simulink model "tg9"  (R2022a)
settings: Solver=ode15s  StartTime=0.0  StopTime=10  MaxStep=0.01  RelTol=1e-3
InitFcn:
  | mecha_param2
  | control_param0
values from neighbouring files (symbols this model uses):
  b0 = 0    [sim_IMMC.m]
  b1 = 1    [sim_IMMC.m]
  back0 = 0    [sim_IMMC.m]
  back1 = 0    [sim_IMMC.m]
  boff = 0    [sim_IMMC.m]
  bon = 0    [sim_IMMC.m]
  c = 0.05    [mecha_param2.m]
  c_jointstop = 0.3 / (pi/180)    (= 17.1887338539)    [mecha_param2.m]
  calctalus = sqrt((L_foot - (DJ1x_foot))^2 + (H_foot-r_cs)^2)    [mecha_param2.m]
  calctoes = sqrt((H_foot-r_cs)^2 + (DJ1x_foot)^2)    [mecha_param2.m]
  corrD = 0.001    [control_param0.m]
  DG_HAT = 0.35    [mecha_param2.m]
  DG_thigh = 0.28    [mecha_param2.m]
  DJ1x_foot = 0.16-r_cs    (= 0.135)    [mecha_param2.m]
  eref = 0.04    [mecha_param2.m]
  FmaxBFSH = 350    [mecha_param2.m]
  FmaxGAS = 1500    [mecha_param2.m]
  FmaxGLU = 1500    [mecha_param2.m]
  FmaxHAM = 3000    [mecha_param2.m]
  FmaxHFL = 2000    [mecha_param2.m]
  FmaxRF = 1200    [mecha_param2.m]
  FmaxSOL = 4000    [mecha_param2.m]
  FmaxTA = 800    [mecha_param2.m]
  FmaxVAS = 6000    [mecha_param2.m]
  g = 9.81    [mecha_param2.m]
  g0 = 0    [sim_IMMC.m]
  g1 = 0    [sim_IMMC.m]
  H_foot = 0.08    [mecha_param2.m]
  In_HAT = 3    [mecha_param2.m]
  In_shank = 0.05    [mecha_param2.m]
  In_thigh = 0.15    [mecha_param2.m]
  K = 5    [mecha_param2.m]
  knee_thigh = [0 0 -(L_thigh/2)]    [mecha_param2.m]
  Kpress = m_HAT * g / DeltaThRef    (= 104967)    [mecha_param2.m]
  L_foot = 0.2    [mecha_param2.m]
  L_HAT = 0.8    [mecha_param2.m]
  L_shank = 0.46    [mecha_param2.m]
  L_thigh = 0.46    [mecha_param2.m]
  LoHAM = table2array(mt('LoHAM', 1))    [control_param0.m]
  LoHFL = table2array(mt('LoHFL', 1))    [control_param0.m]
  longD = longD - corrD    (= 0.019)    [control_param0.m]
  loptBFSH = 0.12    [mecha_param2.m]
  loptGAS = 0.05    [mecha_param2.m]
  loptGLU = 0.11    [mecha_param2.m]
  loptHAM = 0.10    (= 0.1)    [mecha_param2.m]
  loptHFL = 0.11    [mecha_param2.m]
  loptRF = 0.08    [mecha_param2.m]
  loptSOL = 0.04    [mecha_param2.m]
  loptTA = 0.06    [mecha_param2.m]
  loptVAS = 0.08    [mecha_param2.m]
  LoTA = table2array(mt('LoTA', 1))    [control_param0.m]
  lslackBFSH = 0.10    (= 0.1)    [mecha_param2.m]
  lslackGAS = 0.40    (= 0.4)    [mecha_param2.m]
  lslackGLU = 0.13    [mecha_param2.m]
  lslackHAM = 0.31    [mecha_param2.m]
  lslackHFL = 0.10    (= 0.1)    [mecha_param2.m]
  lslackRF = 0.35    [mecha_param2.m]
  lslackSOL = 0.26    [mecha_param2.m]
  lslackTA = 0.24    [mecha_param2.m]
  lslackVAS = 0.23    [mecha_param2.m]
  m_HAT = 53.5    [mecha_param2.m]
  m_shank = 3.5    [mecha_param2.m]
  m_thigh = 8.5    [mecha_param2.m]
  midD = midD - corrD    (= 0.009)    [control_param0.m]
  N = 1.5    [mecha_param2.m]
  nonoff = 0    [control_param0.m]
  phi_a_low = (70) * (pi / 180)    (= 1.2217304764)    [mecha_param2.m]
  phi_a_up = (130) * (pi / 180)    (= 2.26892802759)    [mecha_param2.m]
  phi_dl = 180    [mecha_param2.m]
  phi_h = 230 * (pi / 180)    (= 4.01425727959)    [mecha_param2.m]
  phi_k = 175 * (pi / 180)    (= 3.05432619099)    [mecha_param2.m]
  phictoes = asind((DJ1y_foot-r_cs)/calctoes)    [mecha_param2.m]
  phimaxGASa = 100*pi/180    (= 1.74532925199)    [mecha_param2.m]
  phimaxGASk = 140*pi/180    (= 2.44346095279)    [mecha_param2.m]
  phimaxRFk = 165*pi/180    (= 2.87979326579)    [mecha_param2.m]
  phimaxSOL = 100*pi/180    (= 1.74532925199)    [mecha_param2.m]
  phimaxTA = 80*pi/180    (= 1.3962634016)    [mecha_param2.m]
  phimaxVAS = 165*pi/180    (= 2.87979326579)    [mecha_param2.m]
  phirefBFSH = 160*pi/180    (= 2.79252680319)    [mecha_param2.m]
  phirefGASa = 80*pi/180    (= 1.3962634016)    [mecha_param2.m]
  phirefGASk = 165*pi/180    (= 2.87979326579)    [mecha_param2.m]
  phirefGLU = 120*pi/180    (= 2.09439510239)    [mecha_param2.m]
  phirefHAMh = 150*pi/180    (= 2.61799387799)    [mecha_param2.m]
  phirefHAMk = 180*pi/180    (= 3.14159265359)    [mecha_param2.m]
  phirefHFL = 160*pi/180    (= 2.79252680319)    [mecha_param2.m]
  phirefRFh = 170*pi/180    (= 2.96705972839)    [mecha_param2.m]
  phirefRFk = 125*pi/180    (= 2.18166156499)    [mecha_param2.m]
  phirefSOL = 90*pi/180    (= 1.57079632679)    [mecha_param2.m]
  phirefTA = 110*pi/180    (= 1.91986217719)    [mecha_param2.m]
  phirefVAS = 120*pi/180    (= 2.09439510239)    [mecha_param2.m]
  phiScaleGASa = acos(rGASamin/rGASamax)/(phiminGASa-phimaxGASa)    [mecha_param2.m]
  phiScaleGASk = acos(rGASkmin/rGASkmax)/(phiminGASk-phimaxGASk)    [mecha_param2.m]
  phiScaleRFk = acos(rRFkmin/rRFkmax)/(phiminRFk-phimaxRFk)    [mecha_param2.m]
  phiScaleSOL = acos(rSOLmin/rSOLmax)/(phiminSOL-phimaxSOL)    [mecha_param2.m]
  phiScaleTA = acos(rTAmin/rTAmax)/(phiminTA-phimaxTA)    [mecha_param2.m]
  phiScaleVAS = acos(rVASmin/rVASmax)/(phiminVAS-phimaxVAS)    [mecha_param2.m]
  r1 = 0    [sim_IMMC.m]
  r_cs = 0.025    [mecha_param2.m]
  rBFSH = 0.04    [mecha_param2.m]
  rGASamax = 0.06    [mecha_param2.m]
  rGASkmax = 0.05    [mecha_param2.m]
  rGLU = 0.08    [mecha_param2.m]
  rHAMh = 0.08    [mecha_param2.m]
  rHAMk = 0.05    [mecha_param2.m]
  rHFL = 0.08    [mecha_param2.m]
  rhoBFSH = 0.7    [mecha_param2.m]
  rhoGASa = 0.7    [mecha_param2.m]
  rhoGASk = 0.7    [mecha_param2.m]
  rhoGLU = 0.5    [mecha_param2.m]
  rhoHAMh = 0.5    [mecha_param2.m]
  rhoHAMk = 0.5    [mecha_param2.m]
  rhoHFL = 0.5    [mecha_param2.m]
  rhoRFh = 0.3    [mecha_param2.m]
  rhoRFk = 0.5    [mecha_param2.m]
  rhoSOL = 0.5    [mecha_param2.m]
  rhoTA = 0.7    [mecha_param2.m]
  rhoVAS = 0.6    [mecha_param2.m]
  rRFh = 0.08    [mecha_param2.m]
  rRFkmax = 0.06    [mecha_param2.m]
  rSOLmax = 0.06    [mecha_param2.m]
  ... (+25 more)
undefined symbols (not defined in the file or in its folder): beta11, beta12, beta13, beta14, beta15, beta16, beta21, beta22, beta23, beta24, beta25, beta26, beta31, beta32, beta33, beta34, beta35, beta36, beta41, beta42, beta43, beta44, beta45, beta46, beta51, beta52, beta53, beta54, beta55, beta56, betab1, betab2, betab3, betab4, betab5, betab6, betap11, betap12, betap13, betap14, betap15, betap16, betap21, betap22, betap23, betap24, betap25, betap26, betap31, betap32, betap33, betap34, betap35, betap36, betap41, betap42, betap43, betap44, betap45, betap46 ... (+102)
libraries: sm_lib x89, simulink x72, nesl_utility x58, simulink_extras x18
(part 11 of 12)

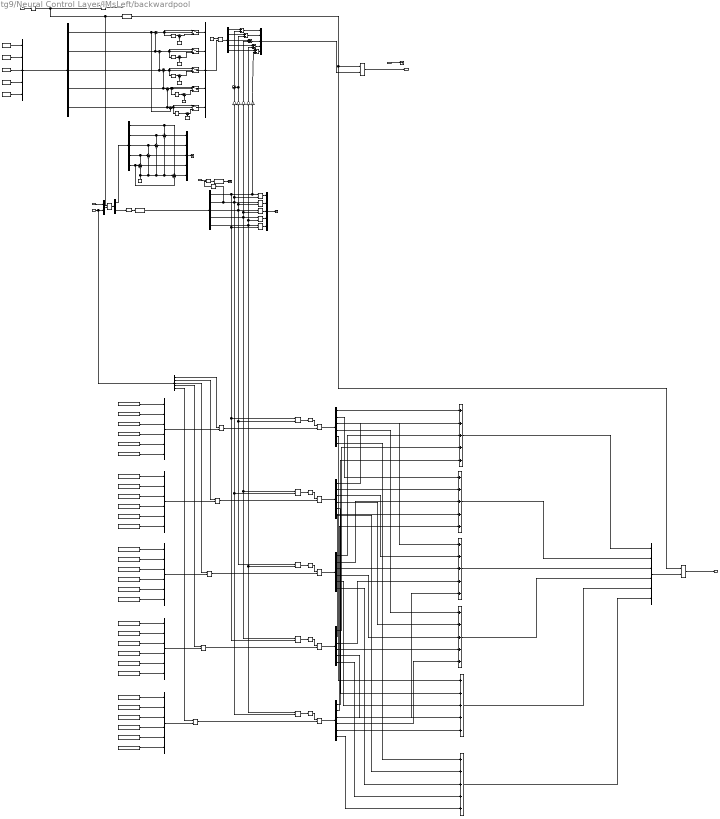
== system tg9/Neural Control Layer/IMsLeft/backwardpool ==
  eta : Inport
  phase : Inport  Port=2
  ui : Inport  Port=3
  right2left : Inport  Port=4
  triggers : Inport  Port=5
  control : Inport  Port=6
  Abs{,1..4} (5 alike) : Abs  ZeroCross=off  SaturateOnIntegerOverflow=off
  Add{,1..4} (5 alike) : Sum
  Add{5,11..15} (6 alike) : Sum  Inputs=+++++
  Cast To Double : DataTypeConversion  OutDataTypeStr=double  SaturateOnIntegerOverflow=off  RndMeth=Floor
  Cast To Double1 : DataTypeConversion  OutDataTypeStr=double  SaturateOnIntegerOverflow=off  RndMeth=Floor
  Cast To Double2 : DataTypeConversion  OutDataTypeStr=double  SaturateOnIntegerOverflow=off  RndMeth=Floor
  Compare To Constant : simulink/Logic and Bit Operations/Compare To Constant  relop=>  const=0.001  OutDataTypeStr=boolean  ZeroCross=off
  Compare To Constant1 : simulink/Logic and Bit Operations/Compare To Constant  relop=<  const=1  OutDataTypeStr=boolean  ZeroCross=off
  Compare To Zero1 : simulink/Logic and Bit Operations/Compare To Zero  relop=>  OutDataTypeStr=boolean  ZeroCross=off
  Constant1 : Constant
  Constant{2,4..6,10} (5 alike) : Constant  Value=2
  Constant3 : Constant  Value=pi
  Demux{,1,4..6} (5 alike) : Demux  Outputs=5
  Demux{8..12} (5 alike) : Demux  Outputs=6
  Demux3 : Demux  Outputs=2
  Divide : Product  Inputs=*/
  Gain{1..4,45} (5 alike) : Gain  Gain=10
  IsPositive{6..10} (5 alike) : simulink/Logic and Bit Operations/Compare To Zero  relop===  OutDataTypeStr=uint8  ZeroCross=off
  Logical Operator : Logic  AllPortsSameDT=off  OutDataTypeStr=boolean
  Mux{1..3,6..7} (5 alike) : Mux  Inputs=5
  Mux{10,16..20} (6 alike) : Mux  Inputs=6
  Mux5 : Mux  Inputs=2
  Product{1..3,6,9,12,17..29,32..36} (24 alike) : Product
  Sum{,1..3,5..6,8..9,11..12} (10 alike) : Sum  Inputs=|-+
  Sum{4,7,10,13} (4 alike) : Sum  Inputs=-+-
  Sum14 : Sum  Inputs=+--
  Sum15 : Sum  Inputs=|++
  Switch{,1..4} (5 alike) : Switch  Criteria=u2 > Threshold  ZeroCross=off  SaturateOnIntegerOverflow=off  InputSameDT=off
  Terminator{,2..4} (4 alike) : Terminator
  betap11 : Constant  Value=betap11
  betap12 : Constant  Value=betap12
  betap13 : Constant  Value=betap13
  betap14 : Constant  Value=betap14
  betap15 : Constant  Value=betap15
  betap16 : Constant  Value=betap16
  betap21 : Constant  Value=betap21
  betap22 : Constant  Value=betap22
  betap23 : Constant  Value=betap23
  betap24 : Constant  Value=betap24
  betap25 : Constant  Value=betap25
  betap26 : Constant  Value=betap26
  betap31 : Constant  Value=betap31
  betap32 : Constant  Value=betap32
  betap33 : Constant  Value=betap33
  betap34 : Constant  Value=betap34
  betap35 : Constant  Value=betap35
  betap36 : Constant  Value=betap36
  betap41 : Constant  Value=betap41
  betap42 : Constant  Value=betap42
  betap43 : Constant  Value=betap43
  betap44 : Constant  Value=betap44
  betap45 : Constant  Value=betap45
  betap46 : Constant  Value=betap46
  betap51 : Constant  Value=betap51
  betap52 : Constant  Value=betap52
  betap53 : Constant  Value=betap53
  betap54 : Constant  Value=betap54
  betap55 : Constant  Value=betap55
  betap56 : Constant  Value=betap56
  theta1 : Constant  Value=thetab1
  theta2 : Constant  Value=thetab2
  theta3 : Constant  Value=thetab3
  theta4 : Constant  Value=thetab4
  theta5 : Constant  Value=thetab5
  vartheta : Outport
  beta : Outport  Port=2
  trigger_out : Outport  Port=3
  wires:
  Sum7/1 -> Mux2/2
  Demux4/4 -> Sum9/1, Sum6/2
  Sum15/1 -> Add/2
  Add2/1 -> Mux7/5
  Switch4/1 -> Mux1/5
  Demux/1 -> Sum14/1, Sum4/1
  Sum3/1 -> Switch/3
  Sum4/1 -> Mux2/1
  Demux/5 -> Sum13/2, Sum14/3
  Abs1/1 -> Sum1/1
  Demux5/4 -> Add4/1
  Mux7/1 -> Product17/2
  Sum8/1 -> Switch3/3
  Sum1/1 -> Switch1/3
  Constant1/1 -> Divide/1
  Sum2/1 -> Abs1/1, Switch1/1, Switch1/2
  Switch/1 -> Mux1/1
  Constant2/1 -> Sum3/2
  Constant5/1 -> Sum5/2
  Demux3/1 -> Demux/1
  Sum11/1 -> Switch4/3
  Abs2/1 -> Sum5/1
  Switch2/1 -> Mux1/3
  Constant3/1 -> Sum14/2, Sum4/3, Sum7/3, Sum10/3, Sum13/3
  Demux4/3 -> Sum2/2, Sum6/1
  Sum12/1 -> Switch4/1, Abs4/1, Switch4/2
  Product2/1 -> Mux3/2
  Sum14/1 -> Mux2/5
  Demux5/1 -> Add/1
  Demux/3 -> Sum7/2, Sum10/1
  Sum5/1 -> Switch2/3
  Compare To Zero1/1 -> Product19/2, Cast To Double2/1, Product18/1
  Product18/1 -> Demux3/1
  Product12/1 -> Mux3/5
  triggers/1 -> Product19/1
  Cast To Double/1 -> Demux1/1
  Demux/2 -> Sum4/2, Sum7/1
  phase/1 -> Mux5/1
  Abs3/1 -> Sum8/1
  Sum6/1 -> Switch2/2, Switch2/1, Abs2/1
  Sum13/1 -> Mux2/4
  Constant6/1 -> Sum11/2
  Logical Operator/1 -> Cast To Double1/1
  ui/1 -> Demux6/1, Mux5/2
  Demux5/3 -> Add3/1
  Demux5/2 -> Add1/1
  Demux5/5 -> Add2/1
  Mux1/1 -> Divide/2
  Demux4/5 -> Sum12/1, Sum9/2
  Demux4/2 -> Sum2/1, Sum/2
  Gain1/1 -> Sum15/2, Add1/2
  Add1/1 -> Mux7/2
  Cast To Double1/1 -> Terminator2/1
  Add/1 -> Mux7/1
  right2left/1 -> Logical Operator/1
  Compare To Constant1/1 -> Logical Operator/2
  Constant4/1 -> Sum1/2
  Demux3/2 -> Compare To Constant/1
  Sum/1 -> Switch/2, Abs/1, Switch/1
  Abs4/1 -> Sum11/1
  eta/1 -> Terminator4/1
  Product1/1 -> Mux3/1
  Mux5/1 -> Product18/2
  Abs/1 -> Sum3/1
  Compare To Constant/1 -> Cast To Double/1
  Switch3/1 -> Mux1/4
  Demux4/1 -> Sum/1, Sum12/2
  Sum9/1 -> Abs3/1, Switch3/2, Switch3/1
  Constant10/1 -> Sum8/2
  Product17/1 -> vartheta/1
  Product9/1 -> Mux3/4
  Divide/1 -> Demux5/1
  Product6/1 -> Mux3/3
  Sum10/1 -> Mux2/3
  Cast To Double2/1 -> Product29/1, Product17/1
  control/1 -> Compare To Zero1/1
  Gain4/1 -> Add2/2
  Product19/1 -> trigger_out/1
  Mux6/1 -> Demux4/1
  Demux/4 -> Sum13/1, Sum10/2
  Switch1/1 -> Mux1/2
  Add3/1 -> Mux7/3
  Add4/1 -> Mux7/4
  Gain2/1 -> Add4/2
  Gain45/1 -> Add3/2
  Mux2/1 -> Terminator/1
  Mux3/1 -> Terminator3/1
  Gain3/1 -> Sum15/1
  theta5/1 -> Mux6/5
  theta4/1 -> Mux6/4
  theta3/1 -> Mux6/3
  theta2/1 -> Mux6/2
  theta1/1 -> Mux6/1
  betap11/1 -> Mux10/1
  Demux1/3 -> Product22/1, Product25/2, Product6/1, Product2/2, Gain1/1
  Demux1/2 -> Product2/1, Product28/2, Product3/2, Product1/2, Gain3/1, Compare To Constant1/1
  Product26/1 -> Demux8/1
  IsPositive7/1 -> Product26/1
  Product25/1 -> IsPositive7/1
  betap12/1 -> Mux10/2
  betap13/1 -> Mux10/3
  betap14/1 -> Mux10/4
  betap16/1 -> Mux10/6
  betap15/1 -> Mux10/5
  Product3/1 -> IsPositive6/1
  IsPositive6/1 -> Product20/1
  Product20/1 -> Demux9/1
  Product21/1 -> Demux10/1
  Mux17/1 -> Product34/2
  IsPositive8/1 -> Product21/1
  Product22/1 -> IsPositive8/1
  Product24/1 -> IsPositive9/1
  IsPositive9/1 -> Product23/1
  Mux18/1 -> Product35/2
  Product23/1 -> Demux11/1
  Product27/1 -> Demux12/1
  Mux19/1 -> Product36/2
  IsPositive10/1 -> Product27/1
  Product28/1 -> IsPositive10/1
  Demux1/1 -> Product24/2, Product25/1, Product12/2, Product1/1, Gain4/1
  Demux1/4 -> Product9/1, Product24/1, Product3/1, Product6/2, Gain45/1
  Demux1/5 -> Product12/1, Product28/1, Product22/2, Product9/2, Gain2/1
  Demux8/1 -> Add5/1
  Demux9/2 -> Add11/2
  Demux10/3 -> Add12/3
  Demux11/4 -> Add13/4
  Demux12/5 -> Add14/5
  Demux8/2 -> Add11/1
  Demux8/3 -> Add12/1
  Demux8/4 -> Add13/1
  Demux8/5 -> Add14/1
  Demux8/6 -> Add15/1
  Demux9/1 -> Add5/2
  Demux9/3 -> Add12/2
  Demux9/4 -> Add13/2
  Demux9/5 -> Add14/2
  Demux9/6 -> Add15/2
  Demux10/1 -> Add5/3
  Demux10/2 -> Add11/3
  Demux10/4 -> Add13/3
  Demux10/5 -> Add14/3
  Demux10/6 -> Add15/3
  Demux11/1 -> Add5/4
  Demux11/2 -> Add11/4
  Demux11/3 -> Add12/4
  Demux11/5 -> Add14/4
  Demux11/6 -> Add15/4
  Demux12/1 -> Add5/5
  Demux12/2 -> Add11/5
  Demux12/3 -> Add12/5
  Demux12/4 -> Add13/5
  Demux12/6 -> Add15/5
  betap21/1 -> Mux16/1
  betap22/1 -> Mux16/2
  betap23/1 -> Mux16/3
  betap24/1 -> Mux16/4
  betap25/1 -> Mux16/5
  betap26/1 -> Mux16/6
  betap31/1 -> Mux17/1
  betap32/1 -> Mux17/2
  betap33/1 -> Mux17/3
  betap34/1 -> Mux17/4
  betap35/1 -> Mux17/5
  betap36/1 -> Mux17/6
  betap41/1 -> Mux18/1
  betap42/1 -> Mux18/2
  betap43/1 -> Mux18/3
  betap44/1 -> Mux18/4
  betap45/1 -> Mux18/5
  betap46/1 -> Mux18/6
  betap56/1 -> Mux19/6
  betap51/1 -> Mux19/1
  betap52/1 -> Mux19/2
  betap53/1 -> Mux19/3
  betap54/1 -> Mux19/4
  betap55/1 -> Mux19/5
  Add5/1 -> Mux20/1
  Add11/1 -> Mux20/2
  Add15/1 -> Mux20/6
  Add13/1 -> Mux20/4
  Add12/1 -> Mux20/3
  Add14/1 -> Mux20/5
  Mux10/1 -> Product32/2
  Product32/1 -> Product26/2
  Demux6/1 -> Product32/1
  Mux16/1 -> Product33/2
  Product33/1 -> Product20/2
  Demux6/2 -> Product33/1
  Product34/1 -> Product21/2
  Demux6/3 -> Product34/1
  Product35/1 -> Product23/2
  Demux6/4 -> Product35/1
  Product36/1 -> Product27/2
  Demux6/5 -> Product36/1
  Mux20/1 -> Product29/2
  Product29/1 -> beta/1

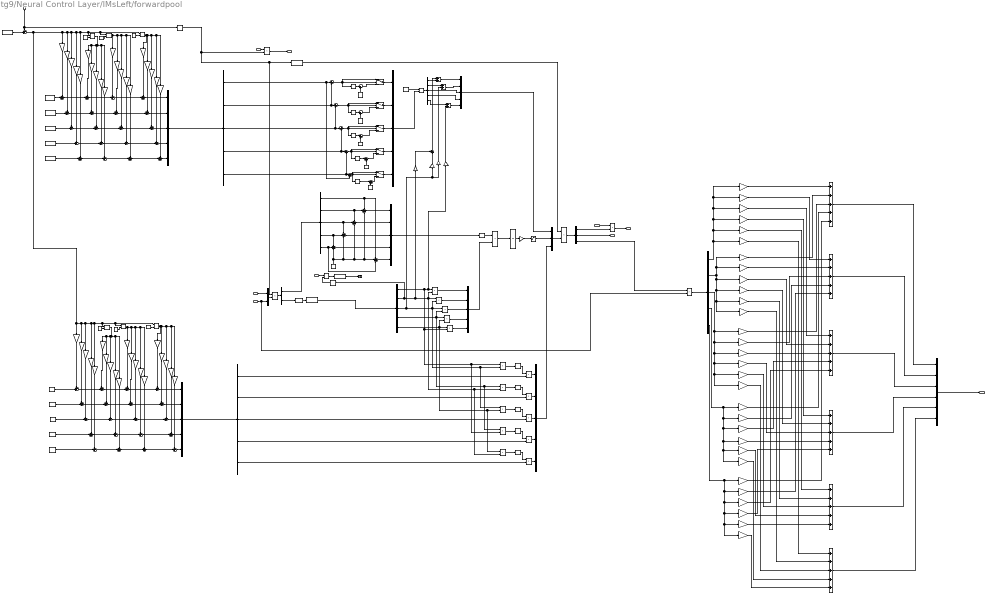
== system tg9/Neural Control Layer/IMsLeft/forwardpool ==
  eta : Inport
  phase : Inport  Port=2
  ui : Inport  Port=3
  right2left : Inport  Port=4
  triggers : Inport  Port=5
  control : Inport  Port=6
  Abs{,1..4} (5 alike) : Abs  ZeroCross=off  SaturateOnIntegerOverflow=off
  Add : Sum
  Add1 : Sum
  Add{6..8,10..12} (6 alike) : Sum  Inputs=+++++
  Add2 : Sum
  Cast To Double : DataTypeConversion  OutDataTypeStr=double  SaturateOnIntegerOverflow=off  RndMeth=Floor
  Cast To Double1 : DataTypeConversion  OutDataTypeStr=double  SaturateOnIntegerOverflow=off  RndMeth=Floor
  Cast To Double2 : DataTypeConversion  OutDataTypeStr=double  SaturateOnIntegerOverflow=off  RndMeth=Floor
  Compare To Constant : simulink/Logic and Bit Operations/Compare To Constant  relop=>  const=0.001  OutDataTypeStr=boolean  ZeroCross=off
  Compare To Constant1 : simulink/Logic and Bit Operations/Compare To Constant  relop=<  const=1  OutDataTypeStr=boolean  ZeroCross=off
  Compare To Zero1 : simulink/Logic and Bit Operations/Compare To Zero  relop=>  OutDataTypeStr=boolean  ZeroCross=off
  Constant1 : Constant
  Constant{2,4..6,10} (5 alike) : Constant  Value=2
  Constant3 : Constant  Value=pi
  Demux{,1,4..5,7,9} (6 alike) : Demux  Outputs=5
  Demux2 : Demux  Outputs=3
  Demux3 : Demux  Outputs=2
  Divide : Product  Inputs=*/
  Gain{,1..4} (5 alike) : Gain  Gain=10
  Gain10 : Gain  Gain=sT42
  Gain11 : Gain  Gain=sT52
  Gain12 : Gain  Gain=sB4
  Gain13 : Gain  Gain=sB5
  Gain14 : Gain  Gain=sB1
  Gain15 : Gain  Gain=sB2
  Gain16 : Gain  Gain=sB3
  Gain17 : Gain  Gain=sB43
  Gain18 : Gain  Gain=sB53
  Gain19 : Gain  Gain=sB13
  Gain20 : Gain  Gain=sT4
  Gain21 : Gain  Gain=sT5
  Gain22 : Gain  Gain=sT1
  Gain23 : Gain  Gain=sT2
  Gain24 : Gain  Gain=sT3
  Gain25 : Gain  Gain=sT43
  Gain26 : Gain  Gain=sT53
  Gain27 : Gain  Gain=sT13
  Gain28 : Gain  Gain=sT23
  Gain29 : Gain  Gain=sT33
  Gain30 : Gain  Gain=sT44
  Gain31 : Gain  Gain=sT54
  Gain32 : Gain  Gain=sT14
  Gain33 : Gain  Gain=sT24
  Gain34 : Gain  Gain=sT34
  Gain35 : Gain  Gain=sB23
  Gain36 : Gain  Gain=sB33
  Gain37 : Gain  Gain=sB44
  Gain38 : Gain  Gain=sB54
  Gain39 : Gain  Gain=sB14
  Gain40 : Gain  Gain=sB24
  Gain41 : Gain  Gain=sB34
  Gain42 : Gain  Gain=sB12
  Gain43 : Gain  Gain=sB22
  Gain44 : Gain  Gain=sB32
  Gain47 : Gain  Gain=beta24
  Gain48 : Gain  Gain=beta14
  Gain49 : Gain  Gain=beta36
  Gain5 : Gain  Gain=sB42
  Gain50 : Gain  Gain=beta13
  Gain51 : Gain  Gain=beta15
  Gain52 : Gain  Gain=beta16
  Gain53 : Gain  Gain=beta12
  Gain54 : Gain  Gain=beta32
  Gain55 : Gain  Gain=beta31
  Gain56 : Gain  Gain=beta46
  Gain57 : Gain  Gain=beta42
  Gain58 : Gain  Gain=beta23
  Gain59 : Gain  Gain=beta41
  Gain6 : Gain  Gain=sB52
  Gain60 : Gain  Gain=beta44
  Gain61 : Gain  Gain=beta43
  Gain62 : Gain  Gain=beta45
  Gain63 : Gain  Gain=beta56
  Gain64 : Gain  Gain=beta52
  Gain65 : Gain  Gain=beta51
  Gain66 : Gain  Gain=beta54
  Gain67 : Gain  Gain=beta53
  Gain68 : Gain  Gain=beta55
  Gain69 : Gain  Gain=beta25
  Gain7 : Gain  Gain=sT12
  Gain71 : Gain  Gain=beta26
  Gain72 : Gain  Gain=beta22
  Gain73 : Gain  Gain=beta21
  Gain74 : Gain  Gain=beta11
  Gain75 : Gain  Gain=beta34
  Gain76 : Gain  Gain=beta33
  Gain77 : Gain  Gain=beta35
  Gain8 : Gain  Gain=sT22
  Gain9 : Gain  Gain=sT32
  Integrator1 : Integrator  ZeroCross=off
  IsPositive{1..5} (5 alike) : simulink/Logic and Bit Operations/Compare To Zero  relop===  OutDataTypeStr=uint8  ZeroCross=off
  Logical Operator : Logic  AllPortsSameDT=off  OutDataTypeStr=boolean
  Mux{,1..3,6..8} (7 alike) : Mux  Inputs=5
  Mux4 : Mux  Inputs=3
  Mux5 : Mux  Inputs=2
  Mux9 : Mux  Inputs=6
  Power{,1..3} (4 alike) : Math  Operator=pow
  Product{1..21} (21 alike) : Product
  Saturation : Saturate  UpperLimit=inf  LowerLimit=0  ZeroCross=off
  Square1 : Math  Operator=pow
  Square2 : Math  Operator=pow
  Sum{,1..3,5..6,8..9,11..12} (10 alike) : Sum  Inputs=|-+
  Sum{4,7,10,13} (4 alike) : Sum  Inputs=-+-
  Sum14 : Sum  Inputs=+--
  Sum{15..16,18..56} (41 alike) : Sum  Inputs=++|
  Sum17 : Sum  Inputs=-+|
  Switch{,1..4} (5 alike) : Switch  Criteria=u2 > Threshold  ZeroCross=off  SaturateOnIntegerOverflow=off  InputSameDT=off
  Terminator2 : Terminator
  Trigonometric Function : Trigonometry
  power1 : Constant  Value=2
  power2 : Constant  Value=3
  power3 : Constant  Value=4
  power4 : Constant  Value=2
  power5 : Constant  Value=3
  power6 : Constant  Value=4
  ref : Constant
  sB01 : Constant  Value=sB01
  sB02 : Constant  Value=sB02
  sB03 : Constant  Value=sB03
  sB04 : Constant  Value=sB04
  sB05 : Constant  Value=sB05
  theta1 : Constant  Value=theta1
  theta2 : Constant  Value=theta2
  theta3 : Constant  Value=theta3
  theta4 : Constant  Value=theta4
  theta5 : Constant  Value=theta5
  phi : Outport
  vartheta : Outport  Port=2
  trigger_out : Outport  Port=3
  beta : Outport  Port=4
  wires:
  Switch1/1 -> Mux1/2
  Demux2/3 -> Product21/1
  Demux/4 -> Sum10/2, Sum13/1
  ref/1 -> Sum17/2
  Product10/1 -> IsPositive3/1
  Mux6/1 -> Demux4/1
  Product19/1 -> trigger_out/1
  Gain4/1 -> Add2/2
  Product8/1 -> Mux/2
  control/1 -> Sum17/1, Compare To Zero1/1
  Sum33/1 -> Sum19/2
  Cast To Double2/1 -> Product17/1
  Sum10/1 -> Mux2/3
  Demux7/2 -> Product8/2
  Sum32/1 -> Sum21/2
  Demux2/2 -> phi/1
  Product15/1 -> IsPositive5/1
  Gain11/1 -> Sum22/1
  Demux1/3 -> Product6/1, Product2/2, Product4/2, Product10/1, Gain2/1, Gain1/1
  Sum36/1 -> Sum18/2
  Product6/1 -> Mux3/3
  Divide/1 -> Demux5/1
  Demux1/2 -> Product1/2, Product7/2, Product15/2, Product2/1, Gain3/1, Compare To Constant1/1
  Product16/1 -> Mux/5
  Product5/1 -> Mux/1
  Sum35/1 -> Sum20/2
  Product9/1 -> Mux3/4
  Product13/1 -> IsPositive4/1
  Product14/1 -> Mux/4
  Product20/1 -> vartheta/1
  Constant10/1 -> Sum8/2
  Sum9/1 -> Switch3/1, Switch3/2, Abs3/1
  Product7/1 -> IsPositive1/1
  IsPositive1/1 -> Product8/1
  Demux4/1 -> Sum12/2, Sum/1
  Switch3/1 -> Mux1/4
  Compare To Constant/1 -> Cast To Double/1
  Abs/1 -> Sum3/1
  Integrator1/1 -> Gain/1
  Mux5/1 -> Product18/2
  Mux/1 -> Mux4/3
  Product17/1 -> Demux2/1
  Product1/1 -> Mux3/1
  Mux4/1 -> Product17/2
  eta/1 -> Product20/1
  Abs4/1 -> Sum11/1
  Gain7/1 -> Sum18/1
  Product3/1 -> Integrator1/1
  Product11/1 -> Mux/3
  Sum/1 -> Switch/1, Abs/1, Switch/2
  Demux3/2 -> Compare To Constant/1
  IsPositive5/1 -> Product16/1
  Constant4/1 -> Sum1/2
  Compare To Constant1/1 -> Logical Operator/2
  right2left/1 -> Logical Operator/1
  Add/1 -> Mux7/1
  Cast To Double1/1 -> Terminator2/1
  Add1/1 -> Mux7/2
  Gain2/1 -> Add1/2
  Demux4/2 -> Sum/2, Sum2/1
  Demux4/5 -> Sum9/2, Sum12/1
  Mux1/1 -> Divide/2
  Demux5/5 -> Add2/1
  Demux5/2 -> Add1/1
  Demux5/3 -> Mux7/3
  ui/1 -> Product21/2, Mux5/2
  Logical Operator/1 -> Cast To Double1/1
  Gain10/1 -> Sum21/1
  Constant6/1 -> Sum11/2
  Sum13/1 -> Mux2/4
  Gain9/1 -> Sum20/1
  Sum6/1 -> Abs2/1, Switch2/1, Switch2/2
  Demux7/5 -> Product16/2
  Abs3/1 -> Sum8/1
  phase/1 -> Mux5/1
  Gain3/1 -> Sum15/1
  Demux/2 -> Sum7/1, Sum4/2
  Trigonometric Function/1 -> Product3/1
  Cast To Double/1 -> Demux1/1
  Demux7/4 -> Product14/2
  Demux7/1 -> Product5/2
  Demux2/1 -> Product20/2
  triggers/1 -> Product19/1
  Product12/1 -> Mux3/5
  Product18/1 -> Demux3/1
  Compare To Zero1/1 -> Product18/1, Cast To Double2/1, Product19/2
  IsPositive4/1 -> Product14/1
  Sum5/1 -> Switch2/3
  Demux/3 -> Sum10/1, Sum7/2
  Demux5/1 -> Add/2
  IsPositive3/1 -> Product11/1
  Sum14/1 -> Mux2/5
  Product2/1 -> Mux3/2
  Mux3/1 -> Product3/2
  Sum12/1 -> Switch4/2, Abs4/1, Switch4/1
  Saturation/1 -> Mux4/2
  Gain1/1 -> Sum15/2
  Demux4/3 -> Sum6/1, Sum2/2
  Mux8/1 -> Demux7/1
  Constant3/1 -> Sum13/3, Sum10/3, Sum7/3, Sum4/3, Sum14/2
  Sum18/1 -> Sum37/2
  Switch2/1 -> Mux1/3
  Abs2/1 -> Sum5/1
  Sum11/1 -> Switch4/3
  Demux3/1 -> Demux/1
  Constant5/1 -> Sum5/2
  Constant2/1 -> Sum3/2
  Switch/1 -> Mux1/1
  Sum2/1 -> Switch1/2, Switch1/1, Abs1/1
  Constant1/1 -> Divide/1
  Sum1/1 -> Switch1/3
  Sum8/1 -> Switch3/3
  Mux7/1 -> Mux4/1
  Demux5/4 -> Mux7/4
  Gain/1 -> Saturation/1
  Abs1/1 -> Sum1/1
  IsPositive2/1 -> Product5/1
  Demux/5 -> Sum14/3, Sum13/2
  Product4/1 -> IsPositive2/1
  Sum4/1 -> Mux2/1
  Sum3/1 -> Switch/3
  Demux/1 -> Sum4/1, Sum14/1
  Switch4/1 -> Mux1/5
  Sum34/1 -> Sum22/2
  Add2/1 -> Mux7/5
  Demux7/3 -> Product11/2
  Gain8/1 -> Sum19/1
  Sum15/1 -> Add/1
  Demux1/5 -> Product12/1, Product10/2, Product15/1, Product9/2
  Demux1/1 -> Gain4/1, Product1/1, Product4/1, Product13/2, Product12/2
  Mux2/1 -> Trigonometric Function/1
  Demux1/4 -> Product9/1, Product7/1, Product13/1, Product6/2
  Demux4/4 -> Sum6/2, Sum9/1
  Sum7/1 -> Mux2/2
  Square1/1 -> Gain10/1, Gain11/1, Gain8/1, Gain7/1, Gain9/1
  Gain22/1 -> Sum36/1
  Gain23/1 -> Sum33/1
  Gain24/1 -> Sum35/1
  Gain20/1 -> Sum32/1
  Gain21/1 -> Sum34/1
  theta1/1 -> Sum36/2
  theta2/1 -> Sum33/2
  theta3/1 -> Sum35/2
  theta4/1 -> Sum32/2
  theta5/1 -> Sum34/2
  power1/1 -> Square1/2
  Sum37/1 -> Sum38/2
  Sum38/1 -> Mux6/1
  Power/1 -> Gain27/1, Gain25/1, Gain26/1, Gain29/1, Gain28/1
  Gain27/1 -> Sum37/1
  power2/1 -> Power/2
  power3/1 -> Power1/2
  Sum39/1 -> Sum40/2
  Sum40/1 -> Mux6/2
  Sum42/1 -> Mux6/3
  Sum41/1 -> Sum42/2
  Sum43/1 -> Sum44/2
  Sum44/1 -> Mux6/4
  Sum19/1 -> Sum39/2
  Gain28/1 -> Sum39/1
  Gain29/1 -> Sum41/1
  Sum20/1 -> Sum41/2
  Gain25/1 -> Sum43/1
  Sum21/1 -> Sum43/2
  Gain26/1 -> Sum45/1
  Sum22/1 -> Sum45/2
  Sum45/1 -> Sum46/2
  Sum46/1 -> Mux6/5
  Gain30/1 -> Sum44/1
  Gain34/1 -> Sum42/1
  Gain33/1 -> Sum40/1
  Gain32/1 -> Sum38/1
  Power1/1 -> Gain30/1, Gain31/1, Gain34/1, Gain33/1, Gain32/1
  Gain31/1 -> Sum46/1
  Sum50/1 -> Mux8/2
  Sum16/1 -> Sum47/2
  Sum54/1 -> Mux8/4
  Sum52/1 -> Mux8/3
  Gain40/1 -> Sum50/1
  Sum25/1 -> Sum53/2
  power6/1 -> Power3/2
  power5/1 -> Power2/2
  Sum56/1 -> Mux8/5
  Power3/1 -> Gain37/1, Gain38/1, Gain41/1, Gain40/1, Gain39/1
  Gain19/1 -> Sum47/1
  Gain18/1 -> Sum55/1
  Sum51/1 -> Sum52/2
  Gain39/1 -> Sum48/1
  Sum23/1 -> Sum49/2
  Sum55/1 -> Sum56/2
  Sum53/1 -> Sum54/2
  Gain36/1 -> Sum51/1
  Sum29/1 -> Sum26/2
  Gain16/1 -> Sum30/1
  Gain15/1 -> Sum28/1
  Sum49/1 -> Sum50/2
  sB02/1 -> Sum28/2
  Gain13/1 -> Sum29/1
  Sum47/1 -> Sum48/2
  Gain14/1 -> Sum31/1
  Gain41/1 -> Sum52/1
  Gain12/1 -> Sum27/1
  sB03/1 -> Sum30/2
  Gain35/1 -> Sum49/1
  Sum30/1 -> Sum24/2
  Sum27/1 -> Sum25/2
  Gain6/1 -> Sum26/1
  Gain44/1 -> Sum24/1
  Gain38/1 -> Sum56/1
  Gain5/1 -> Sum25/1
  Sum48/1 -> Mux8/1
  Sum28/1 -> Sum23/2
  sB05/1 -> Sum29/2
  Sum24/1 -> Sum51/2
  Power2/1 -> Gain19/1, Gain17/1, Gain18/1, Gain36/1, Gain35/1
  Gain17/1 -> Sum53/1
  Gain42/1 -> Sum16/1
  Sum17/1 -> Power3/1, Power2/1, Square2/1, Gain13/1, Gain12/1, Gain16/1, Gain15/1, Gain14/1, Power1/1, Power/1, Square1/1, Gain21/1, Gain20/1, Gain24/1, Gain23/1, Gain22/1
  Gain43/1 -> Sum23/1
  Square2/1 -> Gain5/1, Gain6/1, Gain43/1, Gain42/1, Gain44/1
  power4/1 -> Square2/2
  sB04/1 -> Sum27/2
  Gain37/1 -> Sum54/1
  Sum31/1 -> Sum16/2
  Sum26/1 -> Sum55/2
  sB01/1 -> Sum31/2
  Demux9/4 -> Gain59/1, Gain57/1, Gain61/1, Gain60/1, Gain62/1, Gain56/1
  Demux9/5 -> Gain65/1, Gain64/1, Gain67/1, Gain66/1, Gain68/1, Gain63/1
  Demux9/3 -> Gain55/1, Gain54/1, Gain76/1, Gain75/1, Gain77/1, Gain49/1
  Gain59/1 -> Add12/4
  Gain53/1 -> Add6/1
  Gain54/1 -> Add6/3
  Gain65/1 -> Add12/5
  Gain57/1 -> Add6/4
  Gain64/1 -> Add6/5
  Gain61/1 -> Add7/4
  Demux9/2 -> Gain58/1, Gain71/1, Gain69/1, Gain47/1, Gain73/1, Gain72/1
  Gain67/1 -> Add7/5
  Gain48/1 -> Add8/1
  Gain75/1 -> Add8/3
  Gain66/1 -> Add8/5
  Gain60/1 -> Add8/4
  Gain51/1 -> Add10/1
  Gain62/1 -> Add10/4
  Gain68/1 -> Add10/5
  Gain52/1 -> Add11/1
  Gain50/1 -> Add7/1
  Gain71/1 -> Add11/2
  Gain58/1 -> Add7/2
  Add12/1 -> Mux9/1
  Gain49/1 -> Add11/3
  Gain56/1 -> Add11/4
  Gain77/1 -> Add10/3
  Gain63/1 -> Add11/5
  Gain47/1 -> Add8/2
  Add7/1 -> Mux9/3
  Add8/1 -> Mux9/4
  Add10/1 -> Mux9/5
  Add11/1 -> Mux9/6
  Gain72/1 -> Add6/2
  Gain74/1 -> Add12/1
  Demux9/1 -> Gain74/1, Gain53/1, Gain50/1, Gain48/1, Gain51/1, Gain52/1
  Add6/1 -> Mux9/2
  Gain69/1 -> Add10/2
  Gain55/1 -> Add12/3
  Gain76/1 -> Add7/3
  Gain73/1 -> Add12/2
  Mux9/1 -> beta/1
  Product21/1 -> Demux9/1

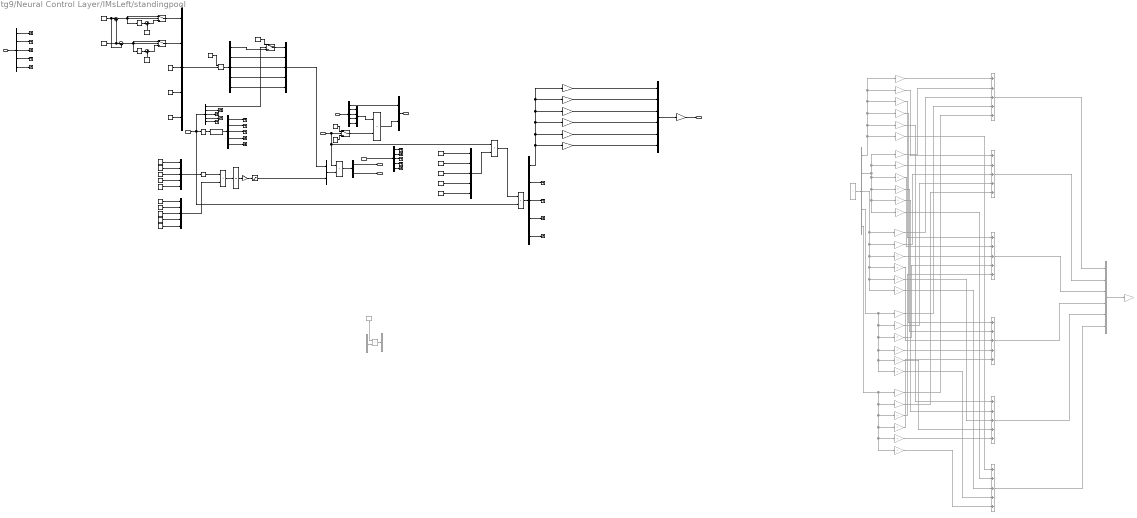
== system tg9/Neural Control Layer/IMsLeft/standingpool ==
  phase : Inport
  ui : Inport  Port=2
  eta : Inport  Port=3
  triggers : Inport  Port=4
  control : Inport  Port=5
  Abs : Abs  ZeroCross=off  SaturateOnIntegerOverflow=off
  Abs1 : Abs  ZeroCross=off  SaturateOnIntegerOverflow=off
  Add{6..8,10..12} (6 alike) : Sum  Commented=on  Inputs=+++++
  Cast To Double : DataTypeConversion  OutDataTypeStr=double  SaturateOnIntegerOverflow=off  RndMeth=Floor
  Compare To Zero : simulink/Logic and Bit Operations/Compare To Zero  relop=>  OutDataTypeStr=boolean  ZeroCross=off
  Compare To Zero1 : simulink/Logic and Bit Operations/Compare To Zero  Commented=on  relop=>  OutDataTypeStr=boolean
  Constant{,3,5..14} (12 alike) : Constant  Value=0
  Constant1 : Constant
  Constant15 : Constant
  Constant2 : Constant  Value=2
  Constant4 : Constant  Value=2
  Demux{,1..2,4,6..8} (7 alike) : Demux  Outputs=5
  Demux3 : Demux  Outputs=2
  Demux5 : Demux  Commented=on  Outputs=2
  Demux9 : Demux  Commented=on  Outputs=5
  Divide : Product  Inputs=*/
  Gain : Gain  Gain=10
  Gain10 : Gain  Gain=beta14
  Gain12 : Gain  Gain=beta13
  Gain13 : Gain  Gain=beta15
  Gain14 : Gain  Gain=beta16
  Gain15 : Gain  Gain=beta12
  Gain31 : Gain
  Gain{32,34,39..58,60..62} (25 alike) : Gain  Commented=on  Gain=0
  Gain33 : Gain  Commented=on  Gain=beta14
  Gain35 : Gain  Commented=on  Gain=beta13
  Gain36 : Gain  Commented=on  Gain=beta15
  Gain37 : Gain  Commented=on  Gain=beta16
  Gain38 : Gain  Commented=on  Gain=beta12
  Gain59 : Gain  Commented=on  Gain=beta11
  Gain64 : Gain  Gain=beta11
  Integrator1 : Integrator  ZeroCross=off
  Mux{,1..4} (5 alike) : Mux  Inputs=5
  Mux11 : Mux  Inputs=6
  Mux5 : Mux  Inputs=2
  Mux6 : Mux  Commented=on  Inputs=2
  Mux7 : Mux
  Mux8 : Mux  Inputs=2
  Mux9 : Mux  Commented=on  Inputs=6
  Product{1..3,5,17} (5 alike) : Product
  Product18 : Product  Commented=on
  Product4 : Product  Commented=on
  Saturation : Saturate  UpperLimit=inf  LowerLimit=0  ZeroCross=off
  Sum{,1..3} (4 alike) : Sum  Inputs=|-+
  Switch : Switch  Criteria=u2 > Threshold  ZeroCross=off  SaturateOnIntegerOverflow=off  InputSameDT=off
  Switch1 : Switch  Criteria=u2 > Threshold  ZeroCross=off  SaturateOnIntegerOverflow=off  InputSameDT=off
  Switch2 : Switch  Criteria=u2 > Threshold  ZeroCross=off  SaturateOnIntegerOverflow=off  InputSameDT=off
  Switch3 : Switch  Threshold=1.98  ZeroCross=off  SaturateOnIntegerOverflow=off  InputSameDT=off
  Terminator{,1..22} (23 alike) : Terminator
  Trigonometric Function : Trigonometry
  nonull1 : Constant  Value=0.5
  null{2..5} (4 alike) : Constant  Value=0
  theta1 : Constant  Value=0
  theta2 : Constant  Value=0.25
  theta3 : Constant
  theta4 : Constant
  theta5 : Constant
  vartheta : Outport
  phi : Outport  Port=2
  beta : Outport  Port=3  InitialOutput=0
  trigger_out : Outport  Port=4
  wires:
  Constant15/1 -> Switch2/3
  Constant/1 -> Switch2/1
  Switch2/1 -> Product1/2
  Mux8/1 -> trigger_out/1
  Product1/1 -> Mux8/2
  Demux6/1 -> Mux8/1
  Mux7/1 -> Product1/1
  Demux6/5 -> Mux7/4
  Demux6/4 -> Mux7/3
  Demux6/3 -> Mux7/2
  Demux6/2 -> Mux7/1
  triggers/1 -> Demux6/1
  Mux6/1 -> Product18/2
  Compare To Zero1/1 -> Product18/1
  Product18/1 -> Demux5/1
  Mux4/1 -> Mux5/1
  Saturation/1 -> Mux5/2
  Demux3/2 -> phi/1
  Mux5/1 -> Product17/2
  Product17/1 -> Demux3/1
  control/1 -> Switch2/2, Product2/1, Product17/1
  Demux4/2 -> Terminator13/1
  Demux4/3 -> Terminator14/1
  Demux4/4 -> Terminator15/1
  Demux4/5 -> Terminator16/1
  Constant14/1 -> Mux3/1
  Constant8/1 -> Mux3/2
  Constant11/1 -> Mux3/3
  Constant12/1 -> Mux3/4
  Constant13/1 -> Mux3/5
  Constant7/1 -> Mux2/5
  Constant6/1 -> Mux2/4
  Constant5/1 -> Mux2/3
  Constant3/1 -> Mux2/2
  Constant9/1 -> Mux2/1
  Demux2/1 -> Switch3/3
  Switch3/1 -> Mux4/1
  Constant10/1 -> Switch3/1
  Demux4/1 -> Switch3/2
  Demux1/5 -> Terminator9/1
  Demux1/4 -> Terminator8/1
  Demux1/3 -> Terminator7/1
  Demux1/2 -> Terminator6/1
  Demux1/1 -> Terminator5/1
  Demux2/5 -> Mux4/5
  Demux2/4 -> Mux4/4
  Demux2/2 -> Mux4/2
  Demux2/3 -> Mux4/3
  Divide/1 -> Demux2/1
  Demux/5 -> Terminator4/1
  Demux/4 -> Terminator3/1
  Demux/3 -> Terminator2/1
  Demux/2 -> Terminator1/1
  Demux/1 -> Terminator/1
  theta5/1 -> Mux1/5
  theta4/1 -> Mux1/4
  Switch1/1 -> Mux1/2
  theta2/1 -> Sum/2, Sum2/1
  Sum3/1 -> Switch/3
  theta3/1 -> Mux1/3
  Abs/1 -> Sum3/1
  Constant4/1 -> Sum1/2
  Sum2/1 -> Abs1/1, Switch1/1, Switch1/2
  Sum1/1 -> Switch1/3
  Constant2/1 -> Sum3/2
  Sum/1 -> Switch/2, Abs/1, Switch/1
  theta1/1 -> Sum/1, Sum2/2
  Switch/1 -> Mux1/1
  Abs1/1 -> Sum1/1
  Mux1/1 -> Divide/2
  Constant1/1 -> Divide/1
  phase/1 -> Demux/1
  Trigonometric Function/1 -> Product3/1
  Mux2/1 -> Trigonometric Function/1
  Mux3/1 -> Product3/2
  Gain/1 -> Saturation/1
  Integrator1/1 -> Gain/1
  Compare To Zero/1 -> Cast To Double/1
  Cast To Double/1 -> Demux1/1
  Product3/1 -> Integrator1/1
  Demux3/1 -> vartheta/1
  eta/1 -> Demux7/1
  Demux7/1 -> Terminator10/1
  Demux7/2 -> Terminator11/1
  Demux7/3 -> Terminator12/1
  Demux7/4 -> Terminator17/1
  Demux7/5 -> Terminator18/1
  Gain64/1 -> Mux11/1
  Gain15/1 -> Mux11/2
  Gain12/1 -> Mux11/3
  Gain10/1 -> Mux11/4
  Gain13/1 -> Mux11/5
  Gain14/1 -> Mux11/6
  ui/1 -> Product5/2, Compare To Zero/1, Demux4/1
  Product5/1 -> Demux8/1
  Mux11/1 -> Gain31/1
  Demux8/1 -> Gain14/1, Gain13/1, Gain10/1, Gain12/1, Gain15/1, Gain64/1
  Gain31/1 -> beta/1
  Demux9/5 -> Gain50/1, Gain49/1, Gain52/1, Gain51/1, Gain53/1, Gain48/1
  Demux9/4 -> Gain44/1, Gain42/1, Gain46/1, Gain45/1, Gain47/1, Gain41/1
  Demux9/3 -> Gain40/1, Gain39/1, Gain61/1, Gain60/1, Gain62/1, Gain34/1
  Demux9/2 -> Gain43/1, Gain56/1, Gain54/1, Gain32/1, Gain58/1, Gain57/1
  Demux9/1 -> Gain59/1, Gain38/1, Gain35/1, Gain33/1, Gain36/1, Gain37/1
  Mux9/1 -> Gain55/1
  Product4/1 -> Demux9/1
  Add11/1 -> Mux9/6
  Add10/1 -> Mux9/5
  Add8/1 -> Mux9/4
  Add7/1 -> Mux9/3
  Add6/1 -> Mux9/2
  Add12/1 -> Mux9/1
  Gain48/1 -> Add11/5
  Gain41/1 -> Add11/4
  Gain34/1 -> Add11/3
  Gain56/1 -> Add11/2
  Gain37/1 -> Add11/1
  Gain53/1 -> Add10/5
  Gain47/1 -> Add10/4
  Gain62/1 -> Add10/3
  Gain54/1 -> Add10/2
  Gain36/1 -> Add10/1
  Gain60/1 -> Add8/3
  Gain45/1 -> Add8/4
  Gain51/1 -> Add8/5
  Gain32/1 -> Add8/2
  Gain33/1 -> Add8/1
  Gain52/1 -> Add7/5
  Gain46/1 -> Add7/4
  Gain43/1 -> Add7/2
  Gain35/1 -> Add7/1
  Gain61/1 -> Add7/3
  Gain49/1 -> Add6/5
  Gain42/1 -> Add6/4
  Gain39/1 -> Add6/3
  Gain57/1 -> Add6/2
  Gain38/1 -> Add6/1
  Gain50/1 -> Add12/5
  Gain44/1 -> Add12/4
  Gain40/1 -> Add12/3
  Gain58/1 -> Add12/2
  Gain59/1 -> Add12/1
  Demux8/2 -> Terminator19/1
  Demux8/3 -> Terminator20/1
  Demux8/4 -> Terminator21/1
  Demux8/5 -> Terminator22/1
  null5/1 -> Mux/5
  null4/1 -> Mux/4
  null3/1 -> Mux/3
  null2/1 -> Mux/2
  nonull1/1 -> Mux/1
  Mux/1 -> Product2/2
  Product2/1 -> Product5/1

== system tg9/Neural Control Layer/IMsRight/IMx3 ==
  ui : Inport
  drivers : Inport  Port=2
  phase : Inport  Port=3
  eta : Inport  Port=4
  Compare To Constant : simulink/Logic and Bit Operations/Compare To Constant  relop=>  const=0.01  OutDataTypeStr=boolean
  Compare To Constant1 : simulink/Logic and Bit Operations/Compare To Constant  relop=<  const=pi  OutDataTypeStr=boolean
  Constant1 : Constant
  Constant2 : Constant
  Demux : Demux  Outputs=3
  Demux1 : Demux  Outputs=3
  Divide : Product  Inputs=*/
  Divide1 : Product  Inputs=*/
  Logical Operator : Logic  AllPortsSameDT=off  OutDataTypeStr=boolean
  Logical Operator1 : Logic  Operator=NOT  AllPortsSameDT=off  OutDataTypeStr=boolean
  Mux1 : Mux  Inputs=6
  Power12 : Math  Operator=pow  SignedPower=on
  Power13 : Math  Operator=pow  SignedPower=on
  Product{1..2,4..12,20,23} (13 alike) : Product
  Sum{,1..6} (7 alike) : Sum  Inputs=+++
  Sum7 : Sum  Inputs=+|+
  Switch1 : Switch  Threshold=1.98  ZeroCross=off  SaturateOnIntegerOverflow=off  InputSameDT=off
  Switch8 : Switch  Criteria=u2 ~= 0  Threshold=0.5  ZeroCross=off  SaturateOnIntegerOverflow=off  InputSameDT=off
  betab1 : Gain  Gain=betab1
  betab2 : Gain  Gain=betab2
  betab3 : Gain  Gain=betab3
  betab4 : Gain  Gain=betab4
  betab5 : Gain  Gain=betab5
  betab6 : Gain  Gain=betab6
  betas1 : Gain  Gain=betas1
  betas2 : Gain  Gain=betas2
  betas3 : Gain  Gain=betas3
  betas4 : Gain  Gain=betas4
  betas5 : Gain  Gain=betas5
  betas6 : Gain  Gain=betas6
  betax1 : Gain  Gain=betax1
  betax2 : Gain  Gain=betax2
  betax3 : Gain  Gain=betax3
  betax4 : Gain  Gain=betax4
  betax5 : Gain  Gain=betax5
  betax6 : Gain  Gain=betax6
  nonact1 : Constant  Value=0
  nonull : Constant  Value=0.5
  null : Constant
  thetab2 : Constant  Value=.25
  thetas2 : Constant  Value=.25
  thetax2 : Constant  Value=thetax
  vartheta : Outport
  beta : Outport  Port=2
  wires:
  betax5/1 -> Sum5/1
  betax6/1 -> Sum6/1
  betax4/1 -> Sum4/1
  betax3/1 -> Sum3/1
  betax2/1 -> Sum2/1
  betax1/1 -> Sum1/1
  betab5/1 -> Sum5/3
  betab4/1 -> Sum4/3
  Sum1/1 -> Mux1/1
  Sum2/1 -> Mux1/2
  Sum3/1 -> Mux1/3
  Sum4/1 -> Mux1/4
  Sum5/1 -> Mux1/5
  Sum6/1 -> Mux1/6
  betab6/1 -> Sum6/3
  betab3/1 -> Sum3/3
  betab2/1 -> Sum2/3
  betab1/1 -> Sum1/3
  betas6/1 -> Sum6/2
  betas4/1 -> Sum4/2
  betas3/1 -> Sum3/2
  betas5/1 -> Sum5/2
  betas2/1 -> Sum2/2
  betas1/1 -> Sum1/2
  Product9/1 -> betas1/1, betas2/1, betas3/1, betas4/1, betas5/1, betas6/1
  Mux1/1 -> beta/1
  Product8/1 -> betax4/1, betax1/1, betax2/1, betax3/1, betax5/1, betax6/1
  Product12/1 -> betab1/1, betab2/1, betab4/1, betab5/1, betab6/1, betab3/1
  Sum/1 -> vartheta/1
  Product7/1 -> Sum/3
  Product6/1 -> Sum/2
  Product4/1 -> Sum/1
  Product20/1 -> Product4/2, Product6/2
  Switch8/1 -> Product9/2, Product8/2
  nonact1/1 -> Switch1/1
  Divide1/1 -> Product2/2
  Switch1/1 -> Product7/2
  ui/1 -> Product5/1, Product1/1, Product12/2
  thetab2/1 -> Divide1/2
  Demux1/3 -> Product2/1
  Product1/1 -> Switch1/2
  Constant2/1 -> Divide1/1
  Product2/1 -> Switch1/3
  Demux/3 -> Product7/1, Product12/1, Product1/2
  Power12/1 -> Product23/2
  Power13/1 -> Product23/1
  Demux1/2 -> Product11/1
  Demux1/1 -> Product10/1
  eta/1 -> Demux1/1
  Product10/1 -> Sum7/1
  Product11/1 -> Sum7/2
  Demux/2 -> Product11/2, Power12/2, Product9/1, Product6/1
  thetas2/1 -> Power12/1
  Demux/1 -> Product10/2, Power13/2, Product4/1, Product8/1
  thetax2/1 -> Power13/1
  drivers/1 -> Demux/1
  Logical Operator1/1 -> Switch8/2
  Logical Operator/1 -> Logical Operator1/1
  Compare To Constant1/1 -> Logical Operator/1
  Compare To Constant/1 -> Logical Operator/2
  phase/1 -> Compare To Constant1/1, Compare To Constant/1
  Product5/1 -> Switch8/1
  null/1 -> Switch8/3
  Divide/1 -> Product20/2
  nonull/1 -> Product5/2
  Constant1/1 -> Divide/1
  Product23/1 -> Divide/2
  Sum7/1 -> Product20/1

== system tg9/Neural Control Layer/IMsRight/S1 ==
  note: Cosine integrator
  phi : Inport
  varthetau : Inport  Port=2
  Enable : EnablePort  StatesWhenEnabling=reset
  Add Constant : Bias  Bias=1  SaturateOnIntegerOverflow=off
  Add Constant3 : Bias  Bias=pi+0.02  SaturateOnIntegerOverflow=off
  Add2 : Sum  Inputs=+++
  Gain1 : Gain  Gain=2*pi
  Integrator1 : Integrator  InitialCondition=0.01  LimitOutput=on  UpperSaturationLimit=1  WrappedStateUpperValue=0  ZeroCross=off
  Product : Product
  Relational Operator : RelationalOperator  OutDataTypeStr=boolean  ZeroCross=off  RndMeth=Simplest  InputSameDT=off
  Terminator : Terminator
  cosine wave : MATLAB Function  TreatAsAtomicUnit=on
  phase : Constant  Value=pi
  phase1 : Constant  Value=0
  u1 : Outport
  theta : Outport  Port=2
  wires:
  phase1/1 -> Add2/3
  phi/1 -> Terminator/1
  varthetau/1 -> Integrator1/1
  Add2/1 -> cosine wave/1(u)
  Gain1/1 -> Relational Operator/2, Add2/1
  Product/1 -> u1/1
  phase/1 -> Add2/2
  Add Constant3/1 -> Relational Operator/1, theta/1
  Integrator1/1 -> Gain1/1
  Relational Operator/1 -> Product/2
  cosine wave/1(y) -> Add Constant/1
  cosine wave/2(theta) -> Add Constant3/1
  Add Constant/1 -> Product/1

== system tg9/Neural Control Layer/IMsRight/S2 ==
  note: Cosine integrator
  varthetau : Inport
  phi : Inport  Port=2
  Enable : EnablePort  StatesWhenEnabling=reset
  Add Constant : Bias  Bias=1  SaturateOnIntegerOverflow=off
  Add Constant3 : Bias  Bias=pi+0.02  SaturateOnIntegerOverflow=off
  Add2 : Sum  Inputs=+++
  Gain1 : Gain  Gain=2*pi
  Integrator1 : Integrator  InitialCondition=0.01  LimitOutput=on  UpperSaturationLimit=1  WrappedStateUpperValue=0  ZeroCross=off
  Product : Product
  Relational Operator : RelationalOperator  OutDataTypeStr=boolean  ZeroCross=off  RndMeth=Simplest  InputSameDT=off
  Terminator : Terminator
  cosine wave : MATLAB Function  TreatAsAtomicUnit=on
  phase : Constant  Value=0
  phase1 : Constant  Value=0
  u2 : Outport
  theta : Outport  Port=2
  wires:
  phase1/1 -> Add2/3
  phi/1 -> Terminator/1
  Product/1 -> u2/1
  cosine wave/1(y) -> Add Constant/1
  cosine wave/2(theta) -> Add Constant3/1
  phase/1 -> Add2/2
  varthetau/1 -> Integrator1/1
  Gain1/1 -> Relational Operator/2, Add2/1
  Relational Operator/1 -> Product/2
  Add2/1 -> cosine wave/1(u)
  Integrator1/1 -> Gain1/1
  Add Constant3/1 -> Relational Operator/1, theta/1
  Add Constant/1 -> Product/1

== system tg9/Neural Control Layer/IMsRight/S3 ==
  note: Cosine integrator
  varthetau : Inport
  phi : Inport  Port=2
  Enable : EnablePort  StatesWhenEnabling=reset
  Add Constant : Bias  Bias=1  SaturateOnIntegerOverflow=off
  Add Constant3 : Bias  Bias=pi+0.02  SaturateOnIntegerOverflow=off
  Add2 : Sum  Inputs=+++
  Gain1 : Gain  Gain=2*pi
  Integrator1 : Integrator  InitialCondition=0.01  LimitOutput=on  UpperSaturationLimit=1  WrappedStateUpperValue=0  ZeroCross=off
  Product : Product
  Relational Operator : RelationalOperator  OutDataTypeStr=boolean  ZeroCross=off  RndMeth=Simplest  InputSameDT=off
  cosine wave : MATLAB Function  TreatAsAtomicUnit=on
  phase : Constant  Value=pi
  u3 : Outport
  theta : Outport  Port=2
  wires:
  Integrator1/1 -> Gain1/1
  Add2/1 -> cosine wave/1(u)
  Relational Operator/1 -> Product/2
  Gain1/1 -> Add2/1, Relational Operator/2
  varthetau/1 -> Integrator1/1
  phase/1 -> Add2/2
  cosine wave/2(theta) -> Add Constant3/1
  cosine wave/1(y) -> Add Constant/1
  Product/1 -> u3/1
  Add Constant3/1 -> Relational Operator/1, theta/1
  Add Constant/1 -> Product/1
  phi/1 -> Add2/3

== system tg9/Neural Control Layer/IMsRight/S4 ==
  note: Cosine integrator
  varthetau : Inport
  phi : Inport  Port=2
  Enable : EnablePort  StatesWhenEnabling=reset
  Add Constant : Bias  Bias=1  SaturateOnIntegerOverflow=off
  Add Constant3 : Bias  Bias=pi+0.02  SaturateOnIntegerOverflow=off
  Add2 : Sum  Inputs=+++
  Gain1 : Gain  Gain=2*pi
  Integrator1 : Integrator  InitialCondition=0.01  LimitOutput=on  UpperSaturationLimit=1  WrappedStateUpperValue=0  ZeroCross=off
  Product : Product
  Relational Operator : RelationalOperator  OutDataTypeStr=boolean  ZeroCross=off  RndMeth=Simplest  InputSameDT=off
  Scope9 : Scope
  cosine wave : MATLAB Function  TreatAsAtomicUnit=on
  phase : Constant  Value=pi
  u3 : Outport
  theta : Outport  Port=2
  wires:
  phi/1 -> Add2/3
  Add Constant/1 -> Product/1
  Add Constant3/1 -> theta/1, Relational Operator/1
  Product/1 -> u3/1
  cosine wave/1(y) -> Add Constant/1
  cosine wave/2(theta) -> Add Constant3/1
  phase/1 -> Add2/2
  varthetau/1 -> Integrator1/1
  Gain1/1 -> Relational Operator/2, Add2/1
  Relational Operator/1 -> Product/2
  Add2/1 -> cosine wave/1(u)
  Integrator1/1 -> Scope9/1, Gain1/1

== system tg9/Neural Control Layer/IMsRight/S5 ==
  note: Cosine integrator
  varthetau : Inport
  phi : Inport  Port=2
  Enable : EnablePort  StatesWhenEnabling=reset
  Add Constant : Bias  Bias=1  SaturateOnIntegerOverflow=off
  Add Constant3 : Bias  Bias=pi+0.02  SaturateOnIntegerOverflow=off
  Add2 : Sum  Inputs=+++
  Gain1 : Gain  Gain=2*pi
  Integrator1 : Integrator  InitialCondition=0.01  LimitOutput=on  UpperSaturationLimit=1  WrappedStateUpperValue=0  ZeroCross=off
  Product : Product
  Relational Operator : RelationalOperator  OutDataTypeStr=boolean  ZeroCross=off  RndMeth=Simplest  InputSameDT=off
  Scope9 : Scope
  Terminator : Terminator
  cosine wave : MATLAB Function  TreatAsAtomicUnit=on
  phase : Constant  Value=pi
  phase1 : Constant  Value=0
  u3 : Outport
  theta : Outport  Port=2
  wires:
  phase1/1 -> Add2/3
  phi/1 -> Terminator/1
  Add2/1 -> cosine wave/1(u)
  Relational Operator/1 -> Product/2
  Gain1/1 -> Add2/1, Relational Operator/2
  varthetau/1 -> Integrator1/1
  phase/1 -> Add2/2
  cosine wave/2(theta) -> Add Constant3/1
  cosine wave/1(y) -> Add Constant/1
  Product/1 -> u3/1
  Add Constant3/1 -> Relational Operator/1, theta/1
  Add Constant/1 -> Product/1
  Integrator1/1 -> Scope9/1, Gain1/1

== system tg9/Neural Control Layer/IMsRight/Sx ==
  note: Cosine integrator
  phi : Inport
  varthetau : Inport  Port=2
  Enable : EnablePort  StatesWhenEnabling=reset
  Add Constant : Bias  Bias=1  SaturateOnIntegerOverflow=off
  Add Constant3 : Bias  Bias=pi+0.02  SaturateOnIntegerOverflow=off
  Add2 : Sum  Inputs=+++
  Gain1 : Gain  Gain=2*pi
  Integrator1 : Integrator  InitialCondition=0.01  LimitOutput=on  UpperSaturationLimit=1  WrappedStateUpperValue=0  ZeroCross=off
  Product : Product
  Relational Operator : RelationalOperator  OutDataTypeStr=boolean  ZeroCross=off  RndMeth=Simplest  InputSameDT=off
  cosine wave : MATLAB Function  TreatAsAtomicUnit=on
  phase : Constant  Value=pi
  u1 : Outport
  theta : Outport  Port=2
  wires:
  Add Constant/1 -> Product/1
  cosine wave/2(theta) -> Add Constant3/1
  cosine wave/1(y) -> Add Constant/1
  Relational Operator/1 -> Product/2
  Integrator1/1 -> Gain1/1
  Add Constant3/1 -> theta/1, Relational Operator/1
  phi/1 -> Add2/3
  phase/1 -> Add2/2
  Product/1 -> u1/1
  Gain1/1 -> Add2/1, Relational Operator/2
  Add2/1 -> cosine wave/1(u)
  varthetau/1 -> Integrator1/1
